simulink model "Ankhbayar_Temuulen_Lab1_Q1"  (R2026a)
settings: Solver=ode45  StopTime=20  MaxStep=1e-3
settings Model: Creator=temuu  LastModifiedBy=temuu

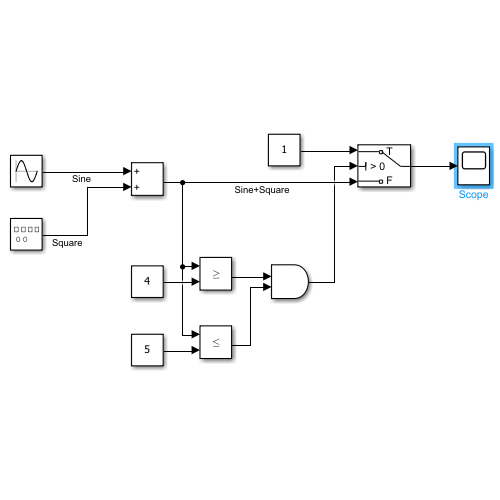
[thumbnail: Simulink's stored preview of the top-level diagram]
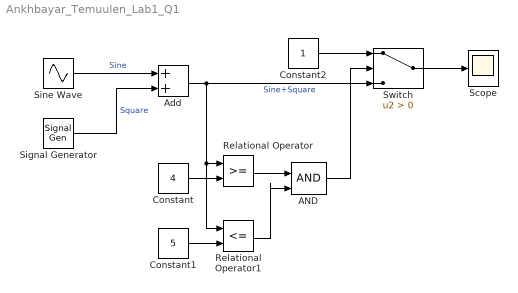
== system Ankhbayar_Temuulen_Lab1_Q1 ==
  AND : Logic  IconShape=distinctive  AllPortsSameDT=off  OutDataTypeStr=boolean
  Add : Sum
  Constant : Constant  Value=4
  Constant1 : Constant  Value=5
  Constant2 : Constant
  Relational Operator : RelationalOperator  OutDataTypeStr=boolean  RndMeth=Simplest  InputSameDT=off
  Relational Operator1 : RelationalOperator  Operator=<=  OutDataTypeStr=boolean  RndMeth=Simplest  InputSameDT=off
  Scope : Scope
      settings: ActiveDisplayYMinimum=-18.021159580184829  ActiveDisplayYMaximum=18.071341613215591
  Signal Generator : SignalGenerator  WaveForm=square  Amplitude=3  Frequency=10  Units=rad/sec
  Sine Wave : Sin  Amplitude=2  SampleTime=0
  Switch : Switch  Criteria=u2 > Threshold  SaturateOnIntegerOverflow=off  InputSameDT=off
  wires:
  Sine Wave/1 -> Add/1  "Sine"
  Signal Generator/1 -> Add/2  "Square"
  Relational Operator/1 -> AND/1
  Relational Operator1/1 -> AND/2
  Constant/1 -> Relational Operator/2
  Constant1/1 -> Relational Operator1/2
  Add/1 -> Switch/3, Relational Operator1/1, Relational Operator/1  "Sine+Square"
  AND/1 -> Switch/2
  Constant2/1 -> Switch/1
  Switch/1 -> Scope/1
